simulink library "angles_lib"  (R2018b)
settings: Solver=VariableStepAuto  StartTime=0.0  StopTime=10.0  RelTol=1e-3
settings Model: Creator=Ybeyer  LastModifiedBy=yannic
settings DebuggingCC: LibraryContextMissingDiagnostic=none
settings SFSimCC: SimUseLocalCustomCode=off
settings RTWCC: RTWUseLocalCustomCode=off
settings CodeAppCC: StateflowObjectComments=on

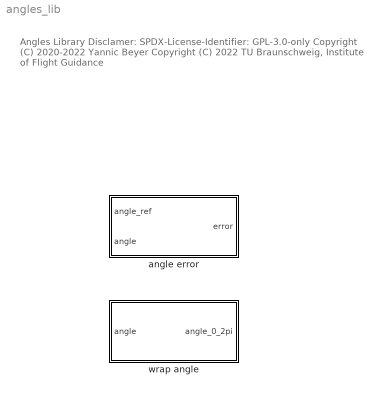
== system angles_lib ==
  note: Angles Library
      |
      | Disclamer:
      | SPDX-License-Identifier: GPL-3.0-only
      |
      | Copyright (C) 2020-2022 Yannic Beyer
      | Copyright (C) 2022 TU Braunschweig, Institute of Flight Guidance
  angle error : MATLAB Function  TreatAsAtomicUnit=on
  wrap angle : MATLAB Function  TreatAsAtomicUnit=on

== matlab function angles_lib/wrap angle ==
  data: angle_0_2pi output; angle input
function angle_0_2pi = fcn(angle) %#codegen
angle_0_2pi = wrapAngle(angle);
end

== matlab function angles_lib/angle error ==
  data: angle_ref input; error output; angle input
function error = fcn(angle_ref,angle) %#codegen
error = errorAngle(angle_ref,angle);
end
